simulink model "Trabajo"  (R2023b)
settings: Solver=VariableStepAuto  StartTime=0.0  StopTime=10.0  RelTol=1e-3
values from neighbouring files (symbols this model uses):
  amp1 = escenarios_dosis(j, 1)    [Trabajo.m]
  amp2 = escenarios_dosis(j, 2)    [Trabajo.m]
  amp3 = escenarios_dosis(j, 3)    [Trabajo.m]
  C50 = P3.C50    [Trabajo.m]
  Gamma = P3.Gamma    [Trabajo.m]
  k10 = P3.k10    [Trabajo.m]
  k12 = P3.k12    [Trabajo.m]
  k13 = P3.k13    [Trabajo.m]
  k1e = 0.456    [Trabajo.m]
  k21 = P3.k21    [Trabajo.m]
  k31 = P3.k31    [Trabajo.m]
  ke0 = 0.456    [Trabajo.m]
  t_off = escenarios_dosis(j, 4)    [Trabajo.m]
settings Model: Creator=anton  LastModifiedBy=anton

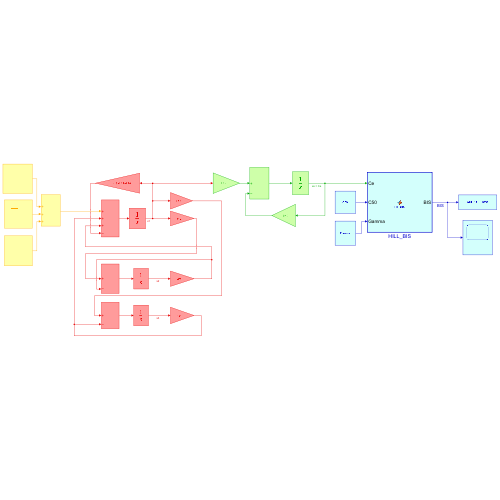
[thumbnail: Simulink's stored preview of the top-level diagram]
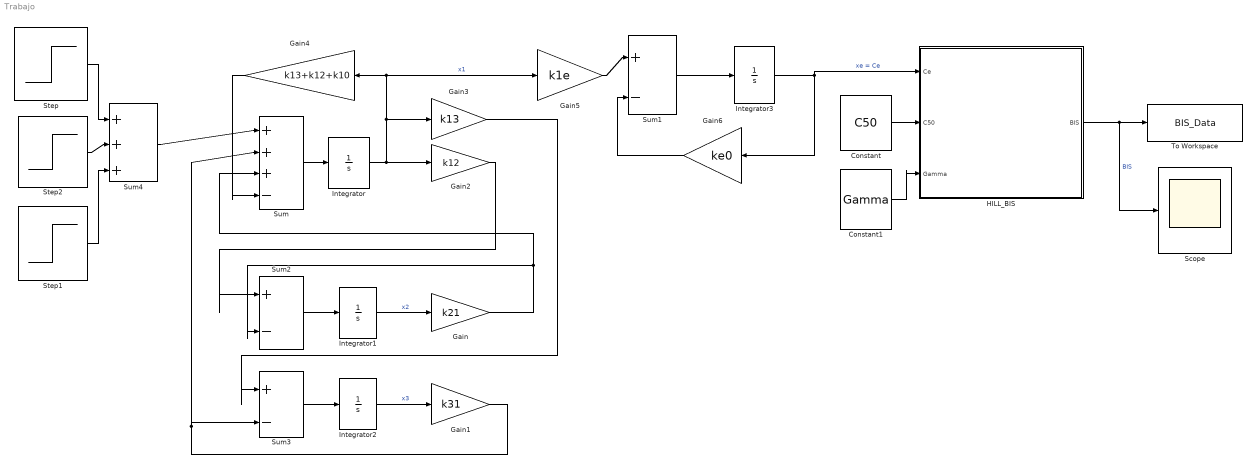
== system Trabajo ==
  Constant : Constant  Value=C50
  Constant1 : Constant  Value=Gamma
  Gain : Gain  Gain=k21
  Gain1 : Gain  Gain=k31
  Gain2 : Gain  Gain=k12
  Gain3 : Gain  Gain=k13
  Gain4 : Gain  Gain=k13+k12+k10
  Gain5 : Gain  Gain=k1e
  Gain6 : Gain  Gain=ke0
  HILL_BIS : MATLAB Function  Tag=Hill_BIS  TreatAsAtomicUnit=on
  Integrator{,1..3} (4 alike) : Integrator
  Scope : Scope
  Step : Step  Time=0  After=amp1  SampleTime=0
  Step1 : Step  Time=t_off  After=amp3  SampleTime=0
  Step2 : Step  Time=t_off  After=amp2  SampleTime=0
  Sum : Sum  Inputs=|+++-
  Sum1 : Sum  Inputs=|+-
  Sum2 : Sum  Inputs=|+-
  Sum3 : Sum  Inputs=|+-
  Sum4 : Sum  Inputs=|+++
  To Workspace : ToWorkspace  VariableName=BIS_Data  SampleTime=-1
  wires:
  Integrator1/1 -> Gain/1  "x2"
  Integrator2/1 -> Gain1/1  "x3"
  Sum/1 -> Integrator/1
  Gain/1 -> Sum/3, Sum2/2
  Gain1/1 -> Sum/2, Sum3/2
  Integrator/1 -> Gain5/1, Gain4/1, Gain3/1, Gain2/1  "x1"
  Sum2/1 -> Integrator1/1
  Gain2/1 -> Sum2/1
  Sum3/1 -> Integrator2/1
  Gain3/1 -> Sum3/1
  Gain4/1 -> Sum/4
  Gain5/1 -> Sum1/1
  Sum1/1 -> Integrator3/1
  Integrator3/1 -> Gain6/1, HILL_BIS/1(Ce)  "xe = Ce"
  Gain6/1 -> Sum1/2
  HILL_BIS/1(BIS) -> Scope/1, To Workspace/1  "BIS"
  Constant/1 -> HILL_BIS/2(C50)
  Constant1/1 -> HILL_BIS/3(Gamma)
  Step/1 -> Sum4/1
  Step2/1 -> Sum4/2
  Step1/1 -> Sum4/3
  Sum4/1 -> Sum/1

== matlab function Trabajo/HILL_BIS ==
  data: Ce input; BIS output; C50 input; Gamma input
function BIS = Hill_BIS(Ce, C50, Gamma)
 
BIS_0 = 100;
BIS_max = 0; 

Ce_pow_gamma = Ce.^Gamma;
C50_pow_gamma = C50.^Gamma;

BIS = BIS_0 + (BIS_max - BIS_0)*(Ce_pow_gamma / (C50_pow_gamma + Ce_pow_gamma));

BIS = max(0, BIS); % Asegurar que el BIS no toma valores negativos

end
